simulink model "mod_qam16"  (R2024b)
settings: Solver=FixedStepDiscrete  StartTime=0.0  StopTime=1  FixedStep=3.1250000000000001e-05  RelTol=1e-3
model workspace (MAT data in the model file):
  M = 16
  Ts = 0.001
  decalage = 0
  df_ol = 1
  fc = 4000
  fs = 32000
  gain_ech = 1.00859371019
  graine = 7
  h_rx = [8.56459526083e-05 0.000117681393507 0.000148802662364 0.000178447986179 0.000206066607265 0.000231128526307 0.000253134118628 0.000271623456863 0.000286185174424 0.000296464708155 0.000302171765366 0.00030308687003 ... (353 elements, 1x353)]
  h_tx = [0.00274067048347 0.00376580459222 0.00476168519565 0.00571033555773 0.00659413143249 0.00739611284184 0.0081002917961 0.00869195061961 0.00915792558158 0.00948687066094 0.00966949649171 0.00969877984097 ... (353 elements, 1x353)]
  ordre = 4
  phi_ol = 0.7
  points = [-1.00155160627-1.00155160627i -1.00155160627-0.333850535422i -1.00155160627+0.333850535422i -1.00155160627+1.00155160627i -0.333850535422-1.00155160627i -0.333850535422-0.333850535422i -0.333850535422+0.333850535422i -0.333850535422+1.00155160627i 0.333850535422-1.00155160627i 0.333850535422-0.333850535422i 0.333850535422+0.333850535422i 0.333850535422+1.00155160627i 1.00155160627-1.00155160627i 1.00155160627-0.333850535422i 1.00155160627+0.333850535422i 1.00155160627+1.00155160627i]
  ptsI = [-1 -1 -1 -1 -0.333333333333 -0.333333333333 -0.333333333333 -0.333333333333 0.333333333333 0.333333333333 0.333333333333 0.333333333333 1 1 1 1]
  ptsQ = [-1 -0.333333333333 0.333333333333 1 -1 -0.333333333333 0.333333333333 1 -1 -0.333333333333 0.333333333333 1 -1 -0.333333333333 0.333333333333 1]
  sigma2 = 0
  sps = 32
  w_boucle = 0.0157079632679
settings Model: Creator=runner  LastModifiedBy=runner

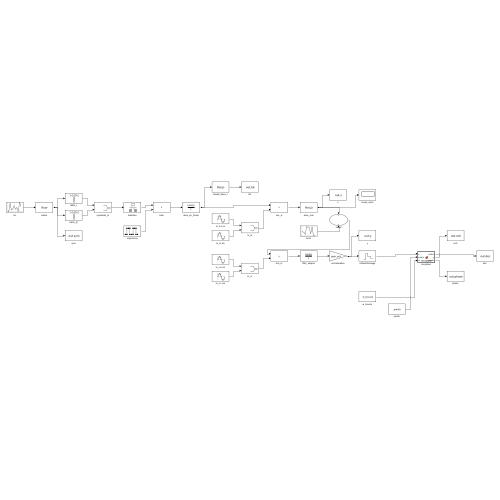
[thumbnail: Simulink's stored preview of the top-level diagram]
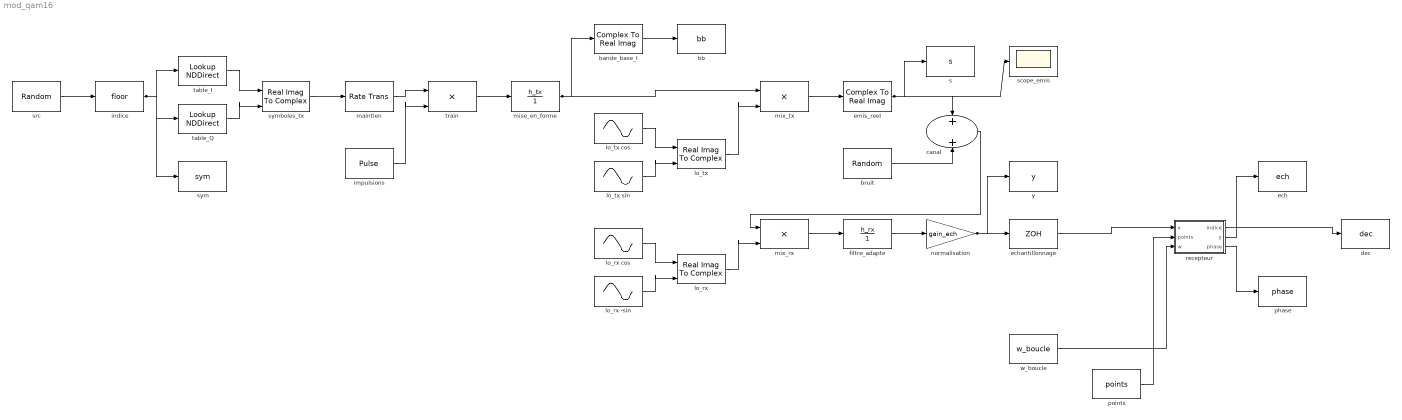
== system mod_qam16 ==
  bande_base_I : ComplexToRealImag  Output=Real
  bb : ToWorkspace  VariableName=bb  SampleTime=-1
  bruit : RandomNumber  Variance=sigma2  Seed=1  SampleTime=1/fs
  canal : Sum
  dec : ToWorkspace  VariableName=dec  SampleTime=-1
  ech : ToWorkspace  VariableName=ech  SampleTime=-1
  echantillonnage : ZeroOrderHold  SampleTime=[Ts, decalage]
  emis_reel : ComplexToRealImag  Output=Real
  filtre_adapte : DiscreteFilter  Numerator=h_rx  Denominator=1
  impulsions : DiscretePulseGenerator  Period=sps  SampleTime=1/fs
  indice : Rounding
  lo_rx : RealImagToComplex
  lo_rx -sin : Sin  Amplitude=-2  Frequency=2*pi*(fc+df_ol)  Phase=phi_ol  SampleTime=1/fs
  lo_rx cos : Sin  Amplitude=2  Frequency=2*pi*(fc+df_ol)  Phase=phi_ol+pi/2  SampleTime=1/fs
  lo_tx : RealImagToComplex
  lo_tx cos : Sin  Frequency=2*pi*fc  Phase=pi/2  SampleTime=1/fs
  lo_tx sin : Sin  Frequency=2*pi*fc  SampleTime=1/fs
  maintien : RateTransition  OutPortSampleTime=1/fs
  mise_en_forme : DiscreteFilter  Numerator=h_tx  Denominator=1
  mix_rx : Product
  mix_tx : Product
  normalisation : Gain  Gain=gain_ech
  phase : ToWorkspace  VariableName=phase  SampleTime=-1
  points : Constant  Value=points
  recepteur : MATLAB Function  TreatAsAtomicUnit=on
  s : ToWorkspace  VariableName=s  SampleTime=-1
  scope_emis : Scope
  src : UniformRandomNumber  Minimum=0  Maximum=M  Seed=graine  SampleTime=Ts
  sym : ToWorkspace  VariableName=sym  SampleTime=-1
  symboles_tx : RealImagToComplex
  table_I : LookupNDDirect  NumberOfTableDimensions=1  Table=ptsI
  table_Q : LookupNDDirect  NumberOfTableDimensions=1  Table=ptsQ
  train : Product
  w_boucle : Constant  Value=w_boucle
  y : ToWorkspace  VariableName=y  SampleTime=-1
  wires:
  src/1 -> indice/1
  indice/1 -> table_I/1, table_Q/1, sym/1
  table_I/1 -> symboles_tx/1
  table_Q/1 -> symboles_tx/2
  symboles_tx/1 -> maintien/1
  maintien/1 -> train/1
  impulsions/1 -> train/2
  train/1 -> mise_en_forme/1
  mise_en_forme/1 -> bande_base_I/1, mix_tx/1
  bande_base_I/1 -> bb/1
  lo_tx cos/1 -> lo_tx/1
  lo_tx sin/1 -> lo_tx/2
  lo_tx/1 -> mix_tx/2
  mix_tx/1 -> emis_reel/1
  emis_reel/1 -> canal/1, s/1, scope_emis/1
  bruit/1 -> canal/2
  lo_rx cos/1 -> lo_rx/1
  lo_rx -sin/1 -> lo_rx/2
  canal/1 -> mix_rx/1
  lo_rx/1 -> mix_rx/2
  mix_rx/1 -> filtre_adapte/1
  filtre_adapte/1 -> normalisation/1
  normalisation/1 -> y/1, echantillonnage/1
  echantillonnage/1 -> recepteur/1(x)
  points/1 -> recepteur/2(points)
  w_boucle/1 -> recepteur/3(w)
  recepteur/2(y) -> ech/1
  recepteur/3(phase) -> phase/1
  recepteur/1(indice) -> dec/1

== matlab function mod_qam16/recepteur ==
  data: indice output; x input; y output; points input; w input; phase output
function [indice, y, phase] = recepteur(x, points, w)
% recepteur de constellation : boucle de phase pilotee par les decisions, comme le bloc
% Constellation Receiver de GNU Radio (erreur = angle entre l'echantillon et le point decide)
persistent ph fr
if isempty(ph), ph = 0; fr = 0; end
z = sqrt(2) / 2; den = 1 + 2 * z * w + w * w; a = 4 * z * w / den; b = 4 * w * w / den;
y = x * exp(-1j * ph); [~, k] = min(abs(y - points)); e = angle(y * conj(points(k)));
fr = fr + b * e; ph = ph + fr + a * e; ph = mod(ph + pi, 2 * pi) - pi; fr = max(-0.1, min(0.1, fr));
indice = k - 1; phase = ph;
end
